simulink model "arduino_serial_comentado_2021_slx"  (R2021a)
settings: Solver=VariableStepAuto  StartTime=0.0  StopTime=inf  RelTol=1e-3
libraries: instrumentseriallib x2
settings Model: Creator=Claudio  LastModifiedBy=mdiaz

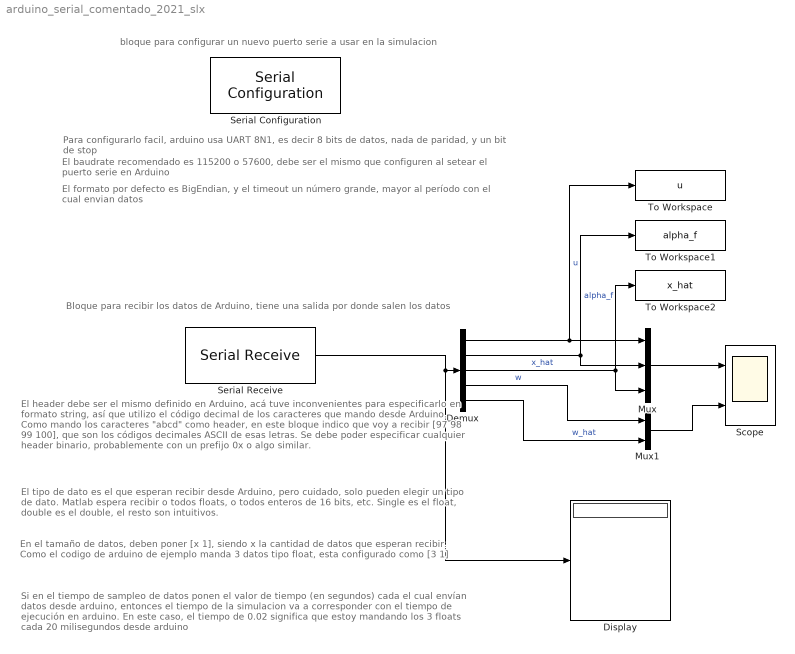
== system arduino_serial_comentado_2021_slx ==
  note: Si en el tiempo de sampleo de datos ponen el valor de tiempo (en segundos) cada el cual envían datos desde arduino, entonces el tiempo de la simulacion va a corresponder con el tiempo de ejecución en arduino. En este caso, el tiempo de 0.02 significa que estoy mandando los 3 floats cada 20 milisegundos desde arduino
  note: En el tamaño de datos, deben poner [x 1], siendo x la cantidad de datos que esperan recibir. Como el codigo de arduino de ejemplo manda 3 datos tipo float, esta configurado como [3 1]
  note: El tipo de dato es el que esperan recibir desde Arduino, pero cuidado, solo pueden elegir un tipo de dato. Matlab espera recibir o todos floats, o todos enteros de 16 bits, etc. Single es el float, double es el double, el resto son intuitivos.
  note: El header debe ser el mismo definido en Arduino, acá tuve inconvenientes para especificarlo en formato string, así que utilizo el código decimal de los caracteres que mando desde Arduino. Como mando los caracteres "abcd" como header, en este bloque indico que voy a recibir [97 98 99 100], que son los códigos decimales ASCII de esas letras. Se debe poder especificar cualquier header binario, probablemente con un prefijo 0x o algo similar.
  note: Bloque para recibir los datos de Arduino, tiene una salida por donde salen los datos
  note: El formato por defecto es BigEndian, y el timeout un número grande, mayor al período con el cual envian datos
  note: El baudrate recomendado es 115200 o 57600, debe ser el mismo que configuren al setear el puerto serie en Arduino
  note: Para configurarlo facil, arduino usa UART 8N1, es decir 8 bits de datos, nada de paridad, y un bit de stop
  note: bloque para configurar un nuevo puerto serie a usar en la simulacion
  Demux : Demux  Outputs=5
  Display : Display
  Mux : Mux  Inputs=3
  Mux1 : Mux  Inputs=2
  Scope : Scope  NumInputPorts=2
  Serial Configuration : instrumentseriallib/Serial Configuration  Priority=-200000  Port=COM4  ComPort=COM4  BaudRate=115200  DataBits=8  Parity=none  StopBits=1  ByteOrder=big-endian  FlowControl=none  Timeout=10  SimulateUsing=Interpreted execution  BlockInModel=on
  Serial Receive : instrumentseriallib/Serial Receive  Priority=1  Port=COM4  ComPort=COM4  DataType=single  SaveDataType=uint8  ToggleHeader=on  Header='abcd'  ToggleTerminator=off  Terminator=<none>  CustomTerminator=[]  ToggleDataSize=on  DataSize=[5 1]  EnableBlockingMode=on  ActionDataUnavailable=Output last received value  ActionWhenDataUnavailable=Output last received value  CustomValue=0  SampleTime=0.02  SimulateUsing=Interpreted execution  BlockInModel=on
  To Workspace : ToWorkspace  VariableName=u  SampleTime=-1
      settings: Save2DSignal=2-D array (concatenate along first dimension)
  To Workspace1 : ToWorkspace  VariableName=alpha_f  SampleTime=-1
      settings: Save2DSignal=2-D array (concatenate along first dimension)
  To Workspace2 : ToWorkspace  VariableName=x_hat  SampleTime=-1
      settings: Save2DSignal=2-D array (concatenate along first dimension)
  wires:
  Demux/2 -> To Workspace1/1, Mux/2  "alpha_f"
  Demux/1 -> To Workspace/1, Mux/1  "u"
  Serial Receive/1 -> Display/1, Demux/1
  Demux/3 -> To Workspace2/1, Mux/3  "x_hat"
  Mux/1 -> Scope/1
  Demux/4 -> Mux1/1  "w"
  Mux1/1 -> Scope/2
  Demux/5 -> Mux1/2  "w_hat"
